simulink model "BuckVoltageControlDemo"  (R2025b)
settings: Solver=ode23t  StartTime=0.0  StopTime=0.25  FixedStep=Ts  MaxStep=1e-4  RelTol=1e-3  EnableMultiTasking=on
PreLoadFcn:
  | BuckVoltageControlData;
undefined symbols (not defined in the file): Ki, Kp, Ts, Tsc
libraries: fl_lib x6, nesl_utility x6, ee_lib x1, eeDcDcVoltageController x1, eePwmGenerator x1
CloseFcn:
  | try,close(h1_BuckVoltageControl),end
  | clear h1_BuckVoltageControl
  | 
  | clear simlog_BuckVoltageControl
  | clear logsout_BuckVoltageControl
Description:
  | Buck Converter Voltage Control
settings Model: Creator=The MathWorks, Inc.  LastModifiedBy=ankur
settings SolverCC: AlgebraicLoopSolver=TrustRegion  MaxZcPerStep=1.0
settings DataIOCC: MaxDataPoints=210000  ReturnWorkspaceOutputs=off  SignalLoggingName=logsout_BuckVoltageControl
settings OptimizationCC: ReuseModelBlockBuffer=off  LifeSpan=inf
settings DebuggingCC: UnconnectedInputMsg=warning  UnconnectedOutputMsg=warning  UnconnectedLineMsg=warning  SubsystemReferenceDiagnosticForUnitTest=warning  SFUnexpectedBacktrackingDiag=warning  SFNoUnconditionalDefaultTransitionDiag=warning  SFExecutionAtInitializationDiag=none  ArithmeticOperatorsInVariantConditions=warning
settings ModelReferenceCC: EnableRefExpFcnMdlSchedulingChecks=on
settings SFSimCC: SimUseLocalCustomCode=off  CustomCodeUndefinedFunction=UseInterfaceOnly
settings RTWCC: RTWUseLocalCustomCode=off  GPUComputeCapability=3.5  DLArmComputeVersion=19.05
settings CodeAppCC: StateflowObjectComments=on
settings GRTTargetCC: TargetLangStandard=C89/C90 (ANSI)
settings ConfigComp: CovMetricSettings=dw  CovSaveCumulativeToWorkspaceVar=on  CovSaveSingleToWorkspaceVar=on  CovExternalEMLEnable=off
settings SimscapeCC: SimscapeNormalizeSystem=off  SimscapeLogType=all  SimscapeLogSimulationStatistics=on  SimscapeLogName=simlog_BuckVoltageControl  SimscapeLogDataHistory=210000.0

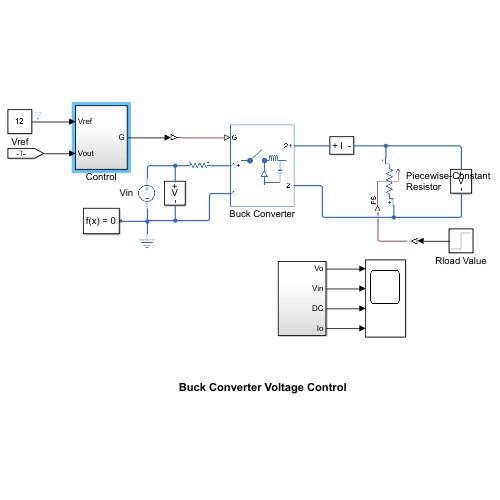
[thumbnail: Simulink's stored preview of the top-level diagram]
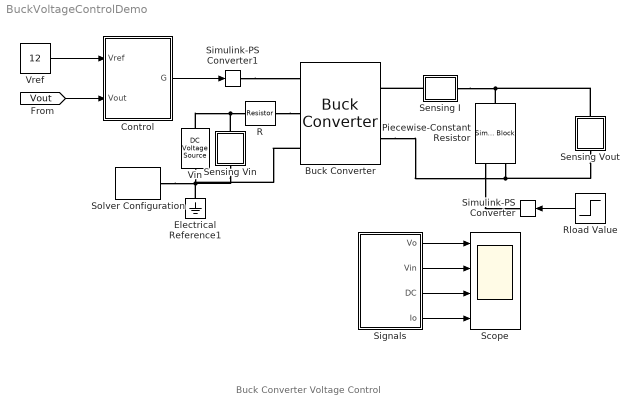
== system BuckVoltageControlDemo ==
  note: Buck Converter Voltage Control
  Buck Converter : ee_lib/Semiconductors & Converters/Converters/Buck Converter  port_option=ee.enum.controlport.ps  device_type=3  Vf=0.8 V  Ron=0.001 Ohm  Rds=0.001 Ohm  Goff=1e-5 1/Ohm  Vgt=1 V  Vgt_off=-1 V  Ih=1 A  Vth=0.5 V  K=0  diode_param=2  diode_Vf=0.8 V  diode_Ron=0.001 Ohm  diode_Goff=1e-5 1/Ohm  diode_C=50 nF  diode_iRM=-235 A  diode_iF=300 A  diode_idot=-50 A/us  diode_trr_param=1  diode_trr_factor=3  diode_trr=15 us  diode_Qrr=1500 s*uA  Lf=L H  Rl=0 Ohm  Cf=C F  Rf=R Ohm  snubber_type=0  Cs=1e-7 F  Rs=0.1 Ohm  iL_specify=off  iL_priority=High  iL=0 A  iL_nominal_specify=off  iL_nominal_value=1  iL_nominal_unit=A  vc_specify=off  vc_priority=High  vc=0 V  vc_nominal_specify=off  vc_nominal_value=1  vc_nominal_unit=V
      settings: InternalSimscapePortConfiguration="{\"Bottom\":[],\"Left\":[{\"id\":\"G\",\"label\":\"G\",\"type\":\"input\"},{\"id\":\"p1\",\"label\":\"1+\",\"type\":\"foundation.electrical.electrical\"},{\"id\":\"n1\",\"label\":\"1-\",\"type\":\"foundation.electrical.electrical\"}],\"Right\":[{\"id\":\"p2\",\"label\":\"2+\",\"type\":\"foundation.electrical.electrical\"},{\"id\":\"n2\",\"label\":\"2-\",\"type\":\"foundation.electrical.electrical\"}],\"Top\":[]}"
  Control : Subsystem
  Electrical Reference1 : fl_lib/Electrical/Electrical Elements/Electrical Reference
  Piecewise-Constant Resistor : SimscapeComponentBlock  SourceFile=PiecewiseConstantResistor  ComponentPath=PiecewiseConstantResistor  ComponentVariants="[\"PiecewiseConstantResistor\"]"  ComponentVariantNames="[\"PiecewiseConstantResistor\"]"  ClassName=PiecewiseConstantResistor  SchemaVersion=1  Rmin=1e-6 Ohm  Rtol=1e-6 Ohm  i_specify=off  i_priority=None  i=0 A  i_nominal_specify=off  i_nominal_value=1  i_nominal_unit=A  v_specify=off  v_priority=None  v=0 V  v_nominal_specify=off  v_nominal_value=1  v_nominal_unit=V
      settings: CopyFcn=simscape.sscblock.internal.componentBlockCallback(gcbh,'COPY')  PreCopyFcn=simscape.sscblock.internal.componentBlockCallback(gcbh,'PRECOPY')  PreDeleteFcn=simscape.sscblock.internal.componentBlockCallback(gcbh,'PREDELETE')  InternalSimscapePortConfiguration="{\"Bottom\":[],\"Left\":[{\"id\":\"R\",\"label\":\"PS\",\"type\":\"input\"},{\"id\":\"p\",\"label\":\"+\",\"type\":\"foundation.electrical.electrical\"}],\"Right\":[{\"id\":\"n\",\"label\":\"-\",\"type\":\"foundation.electrical.electrical\"}],\"Top\":[]}"
      mask Type: Piecewise-Constant Resistor
  R : fl_lib/Electrical/Electrical Elements/Resistor  R=0.001 Ohm  i_specify=off  i_priority=None  i=0 A  i_nominal_specify=off  i_nominal_value=1  i_nominal_unit=A  v_specify=off  v_priority=None  v=0 V  v_nominal_specify=off  v_nominal_value=1  v_nominal_unit=V
  Rload Value : Step  Time=0.15  Before=2  After=3  SampleTime=0
  Scope : Scope  NumInputPorts=4
      settings: ActiveDisplayYMinimum=-2.1925555895835989  ActiveDisplayYMaximum=19.733000307247387
  Sensing Vin : Subsystem
      mask Display:
      | disp('V')
      | port_label('Lconn',1,'+')
      | port_label('Rconn',1,'-')
  Sensing Vout : Subsystem
      mask Display:
      | disp('V')
      | port_label('Lconn',1,'+')
      | port_label('Rconn',1,'-')
  Sensing I : Subsystem
      mask Display:
      | disp('I')
      | port_label('Lconn',1,'+')
      | port_label('Rconn',1,'-')
  Signals : Subsystem
  Simulink-PS Converter : nesl_utility/Simulink-PS Converter  PhysicalDomain=network_engine_domain  SubClassName=ps_input  LeftPortType=input  RightPortType=output  PseudoPeriodic=off  Frequencies=[]  NoiseDistribution=none  NoiseParameters=[]  Unit=1  AffineConversion=off  FilteringAndDerivatives=zero  SimscapeFilterOrder=1  InputFilterTimeConstant=0.001  UdotUserProvided=0
  Simulink-PS Converter1 : nesl_utility/Simulink-PS Converter  PhysicalDomain=network_engine_domain  SubClassName=ps_input  LeftPortType=input  RightPortType=output  PseudoPeriodic=off  Frequencies=[]  NoiseDistribution=none  NoiseParameters=[]  Unit=1  AffineConversion=off  FilteringAndDerivatives=provide  SimscapeFilterOrder=1  InputFilterTimeConstant=0.001  UdotUserProvided=0
  Solver Configuration : nesl_utility/Solver Configuration  PhysicalDomain=network_engine_domain  SubClassName=solver  LeftPortType=input  RightPortType=generic  Tones=[]  Harmonics=[]  SimulateNoise=off  Profile=off  UseLocalSampling=off  EnableSwitchedLinearOptims=on  FrequencyDomain=off  UseCCode=off  RelTol=0.001  AbsTol=1e-06  MinStep=1e-09  ToWorkspace=off  RevertToSquareIcSolve=off  NumHomotopyIterations=100  PhasorMode=off  PhasorModeNumHarmonics=1  ConsistencySolver=NEWTON_FTOL  IndexReductionMethod=DerivativeReplacement  DoDC=off  ResidualTolerance=1e-9  ConsistencyTolSource=GLOBAL  ConsistencyAbsTol=0.001  ConsistencyRelTol=0.001  ConsistencyTolFactor=0.001  UseLocalSolver=on  LocalSolverChoice=NE_BACKWARD_EULER_ADVANCER  ResolveIndetEquations=on  FunctionEvalNumThread=1  LocalSolverSampleTime=Ts  DoFixedCost=on  MaxNonlinIter=3  MaxModeIter=2  ComputeImpulses=off  ImpulseIterations=2  LinearAlgebra=auto  LinearAlgebraNumThread=0  EquationFormulation=NE_TIME_EF  DelaysMemoryBudget=1024  AutomaticFiltering=on  FilteringTimeConstant=0.001  PartitionStorageMethod=AS_NEEDED  PartitionMemoryBudget=1024  PartitionMethod=FAST  MultibodyUseLocalSolver=off  MultibodyLocalSolverChoice=ODE1  MultibodyLocalSolverSampleTime=0.001
  Vin : fl_lib/Electrical/Electrical Sources/DC Voltage Source  v0=Vin15 V
  Vref : Constant  Value=12  SampleTime=Ts
  wires:
  [Vout] -> Control/2(Vout)
  Vref/1 -> Control/1(Vref)
  Control/1(G) -> Simulink-PS Converter1/1
  Rload Value/1 -> Simulink-PS Converter/1
  Signals/1(Vo) -> Scope/1
  Signals/4(Io) -> Scope/4
  Signals/2(Vin) -> Scope/2
  Signals/3(DC) -> Scope/3
  connections:
  Electrical Reference1/LConn1 -- Solver Configuration/RConn1 -- Vin/RConn1 -- Sensing Vin/RConn1 -- Buck Converter/LConn3
  Sensing I/RConn1 -- Piecewise-Constant Resistor/RConn1 -- Sensing Vout/LConn1
  Buck Converter/RConn2 -- Piecewise-Constant Resistor/LConn2 -- Sensing Vout/RConn1
  R/RConn1 -- Buck Converter/LConn2
  Sensing I/LConn1 -- Buck Converter/RConn1
  Piecewise-Constant Resistor/LConn1 -- Simulink-PS Converter/RConn1
  Simulink-PS Converter1/RConn1 -- Buck Converter/LConn1
  Vin/LConn1 -- Sensing Vin/LConn1 -- R/LConn1

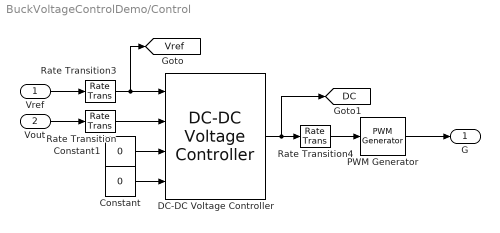
== system BuckVoltageControlDemo/Control ==
  Vref : Inport
  Vout : Inport  Port=2
  Constant : Constant  Value=0
  Constant1 : Constant  Value=0
  DC-DC Voltage Controller : eeDcDcVoltageController/DC-DC Voltage Controller  Kp=Kp  Ki=Ki  Kaw=1  upperLimit=0.95  lowerLimit=0  Ts=Tsc  Tf=0.001  ActVdcFilter=off
  PWM Generator : eePwmGenerator/PWM Generator  CarrCount=Up  Tper=1e-4  Tdelay=0  Ts=Ts
  Rate Transition : RateTransition  OutPortSampleTime=Tsc
  Rate Transition3 : RateTransition  OutPortSampleTime=Tsc
  Rate Transition4 : RateTransition  OutPortSampleTime=Ts
  G : Outport  VectorParamsAs1DForOutWhenUnconnected=off
  tag scope: DC=global, Vref=global
  wires:
  Vref/1 -> Rate Transition3/1
  Rate Transition3/1 -> [Vref], DC-DC Voltage Controller/1
  Vout/1 -> Rate Transition/1
  PWM Generator/1 -> G/1
  DC-DC Voltage Controller/1 -> Rate Transition4/1, [DC]
  Rate Transition4/1 -> PWM Generator/1
  Constant1/1 -> DC-DC Voltage Controller/3
  Constant/1 -> DC-DC Voltage Controller/4
  Rate Transition/1 -> DC-DC Voltage Controller/2

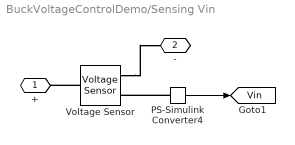
== system BuckVoltageControlDemo/Sensing Vin ==
  PS-Simulink Converter4 : nesl_utility/PS-Simulink Converter  PhysicalDomain=network_engine_domain  SubClassName=ps_output  LeftPortType=input  RightPortType=output  PseudoPeriodic=off  Frequencies=[]  VectorFormat=1-D array  Unit=V  AffineConversion=off
  Voltage Sensor : fl_lib/Electrical/Electrical Sensors/Voltage Sensor
  + : PMIOPort  Side=Left
  - : PMIOPort  Port=2  Side=Right
  tag scope: Vin=global
  wires:
  PS-Simulink Converter4/1 -> [Vin]
  connections:
  PS-Simulink Converter4/LConn1 -- Voltage Sensor/RConn1
  Voltage Sensor/RConn2 -- -/RConn1
  Voltage Sensor/LConn1 -- +/RConn1

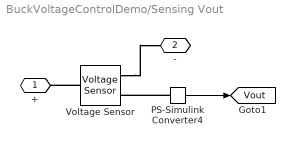
== system BuckVoltageControlDemo/Sensing Vout ==
  PS-Simulink Converter4 : nesl_utility/PS-Simulink Converter  PhysicalDomain=network_engine_domain  SubClassName=ps_output  LeftPortType=input  RightPortType=output  PseudoPeriodic=off  Frequencies=[]  VectorFormat=1-D array  Unit=V  AffineConversion=off
  Voltage Sensor : fl_lib/Electrical/Electrical Sensors/Voltage Sensor
  + : PMIOPort  Side=Left
  - : PMIOPort  Port=2  Side=Right
  tag scope: Vout=global
  wires:
  PS-Simulink Converter4/1 -> [Vout]
  connections:
  Voltage Sensor/LConn1 -- +/RConn1
  Voltage Sensor/RConn2 -- -/RConn1
  PS-Simulink Converter4/LConn1 -- Voltage Sensor/RConn1

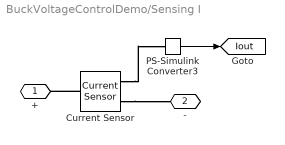
== system BuckVoltageControlDemo/Sensing I ==
  Current Sensor : fl_lib/Electrical/Electrical Sensors/Current Sensor
  PS-Simulink Converter3 : nesl_utility/PS-Simulink Converter  PhysicalDomain=network_engine_domain  SubClassName=ps_output  LeftPortType=input  RightPortType=output  PseudoPeriodic=off  Frequencies=[]  VectorFormat=1-D array  Unit=A  AffineConversion=off
  + : PMIOPort  Side=Left
  - : PMIOPort  Port=2  Side=Right
  tag scope: Iout=global
  wires:
  PS-Simulink Converter3/1 -> [Iout]
  connections:
  Current Sensor/RConn2 -- -/RConn1
  Current Sensor/LConn1 -- +/RConn1
  Current Sensor/RConn1 -- PS-Simulink Converter3/LConn1

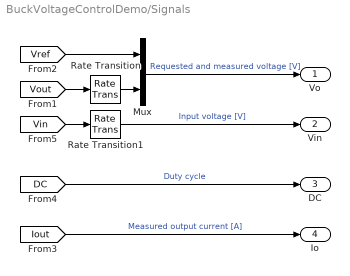
== system BuckVoltageControlDemo/Signals ==
  Mux : Mux  Inputs=2
  Rate Transition : RateTransition  OutPortSampleTime=Tsc
  Rate Transition1 : RateTransition  OutPortSampleTime=Tsc
  Vo : Outport  VectorParamsAs1DForOutWhenUnconnected=off
  Vin : Outport  Port=2  VectorParamsAs1DForOutWhenUnconnected=off
  DC : Outport  Port=3  VectorParamsAs1DForOutWhenUnconnected=off
  Io : Outport  Port=4  VectorParamsAs1DForOutWhenUnconnected=off
  wires:
  [Vout] -> Rate Transition/1
  [Vin] -> Rate Transition1/1
  Rate Transition1/1 -> Vin/1  "Input voltage [V]"
  Mux/1 -> Vo/1  "Requested and measured voltage [V]"
  [Iout] -> Io/1  "Measured output current [A]"
  [Vref] -> Mux/1
  Rate Transition/1 -> Mux/2
  [DC] -> DC/1  "Duty cycle"
